simulink model "E2_ِDifferenceEquation_DT"  (R2024a)
settings: Solver=VariableStepAuto  StartTime=0.0  StopTime=10.0  RelTol=1e-3
settings Model: Creator=Sanagostar  LastModifiedBy=Sanagostar

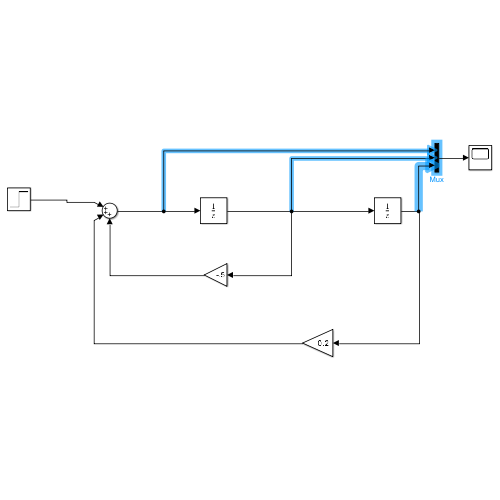
[thumbnail: Simulink's stored preview of the top-level diagram]
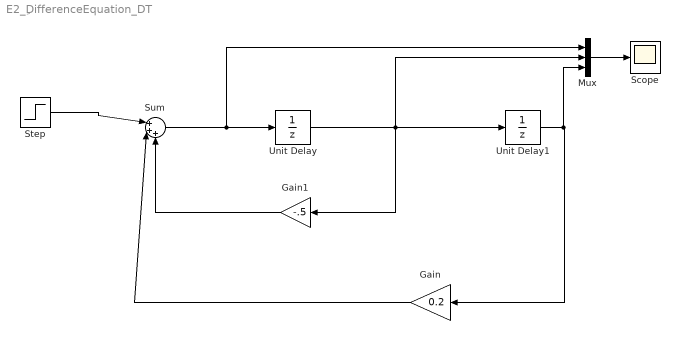
== system E2_ِDifferenceEquation_DT ==
  Gain : Gain  Gain=0.2
  Gain1 : Gain  Gain=-.5
  Mux : Mux  Inputs=3
  Scope : Scope
  Step : Step  SampleTime=0
  Sum : Sum  Inputs=|+++
  Unit Delay : UnitDelay  SampleTime=-1  HasFrameUpgradeWarning=on
  Unit Delay1 : UnitDelay  SampleTime=-1  HasFrameUpgradeWarning=on
  wires:
  Step/1 -> Sum/1
  Sum/1 -> Mux/1, Unit Delay/1
  Unit Delay/1 -> Mux/2, Gain1/1, Unit Delay1/1
  Gain1/1 -> Sum/3
  Unit Delay1/1 -> Mux/3, Gain/1
  Gain/1 -> Sum/2
  Mux/1 -> Scope/1
